simulink model "case_04_slow_to_fast"  (R2025b)
settings: Solver=VariableStepAuto  StartTime=0.0  StopTime=60  RelTol=1e-3
settings Model: Creator=sanborkl  LastModifiedBy=sanborkl

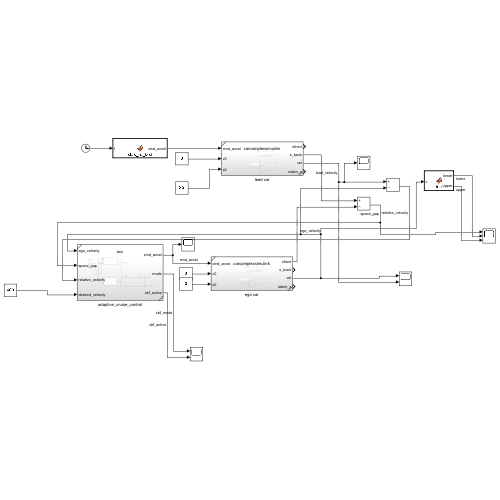
[thumbnail: Simulink's stored preview of the top-level diagram]
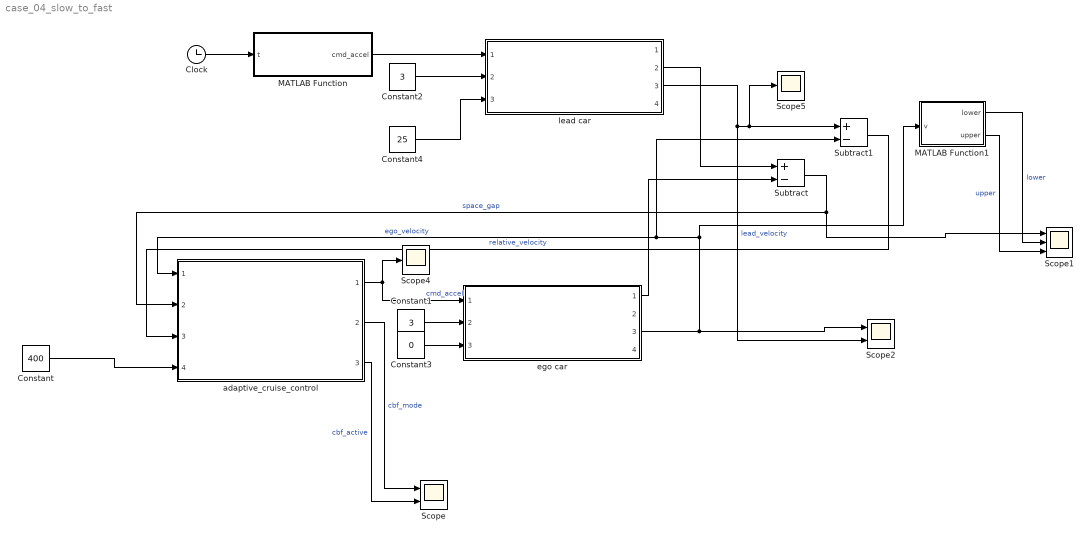
== system case_04_slow_to_fast ==
  Clock : Clock
  Constant : Constant  Value=400
  Constant1 : Constant  Value=3
  Constant2 : Constant  Value=3
  Constant3 : Constant  Value=0
  Constant4 : Constant  Value=25
  MATLAB Function : MATLAB Function  TreatAsAtomicUnit=on
  MATLAB Function1 : MATLAB Function  TreatAsAtomicUnit=on
  Scope : Scope  NumInputPorts=2
      settings: ActiveDisplayYMinimum=0.75000000000000011  ActiveDisplayYMaximum=3.25
  Scope1 : Scope  NumInputPorts=3
      settings: ActiveDisplayYMinimum=1.4597803310159403  ActiveDisplayYMaximum=96.73995170288805  YLabel=m
  Scope2 : Scope  NumInputPorts=2
      settings: ActiveDisplayYMinimum=-1.3046371711049463  ActiveDisplayYMaximum=41.708142832386393  YLabel=m/s  DataLoggingVariableName=ScopeData2
  Scope4 : Scope
      settings: ActiveDisplayYMinimum=-0.20100000000000007  ActiveDisplayYMaximum=1.689  YLabel=m/s^2  DataLoggingVariableName=ScopeData4
  Scope5 : Scope
      settings: ActiveDisplayYMinimum=2.9820782097107514  ActiveDisplayYMaximum=11.601301242824333  YLabel=m/s  DataLoggingVariableName=ScopeData6
  Subtract : Sum  Inputs=+-
  Subtract1 : Sum  Inputs=+-
  adaptive_cruise_control : Subsystem  ReferencedSubsystem=acc
  ego car : Subsystem  ReferencedSubsystem=carcomplexsimulink
  lead car : Subsystem  ReferencedSubsystem=carcomplexsimulink
  wires:
  Subtract/1 -> Scope1/1, adaptive_cruise_control/2  "space_gap"
  MATLAB Function/1(cmd_accel) -> lead car/1
  Constant1/1 -> ego car/2
  MATLAB Function1/2(upper) -> Scope1/3  "upper"
  Subtract1/1 -> adaptive_cruise_control/3  "relative_velocity"
  Clock/1 -> MATLAB Function/1(t)
  Constant2/1 -> lead car/2
  lead car/3 -> Scope2/2, Scope5/1, Subtract1/1  "lead_velocity"
  adaptive_cruise_control/2 -> Scope/1  "cbf_mode"
  ego car/1 -> Subtract/2
  lead car/2 -> Subtract/1
  MATLAB Function1/1(lower) -> Scope1/2  "lower"
  Constant4/1 -> lead car/3
  adaptive_cruise_control/1 -> ego car/1, Scope4/1  "cmd_accel"
  Constant/1 -> adaptive_cruise_control/4
  adaptive_cruise_control/3 -> Scope/2  "cbf_active"
  Constant3/1 -> ego car/3
  ego car/3 -> Subtract1/2, adaptive_cruise_control/1, MATLAB Function1/1(v), Scope2/1  "ego_velocity"

== matlab function case_04_slow_to_fast/MATLAB Function ==
  data: t input; cmd_accel output
function cmd_accel = slow_to_fast(t)

if t < 20
    cmd_accel = sin(0.125*t);
else
    cmd_accel = 0.5;
end

== matlab function case_04_slow_to_fast/MATLAB Function1 ==
  data: v input; lower output; upper output
function [lower, upper] = fcn(v)

lower = 2 * v + 5;
upper = 2 * v + 15;
